simulink model "sm_wheel_loader_vehicle"  (R2025a)
settings: Solver=ode23t  StartTime=0.0  StopTime=70  RelTol=1e-3  AbsTol=1e-3  EnableMultiTasking=on
PostLoadFcn:
  | sm_wheel_loader_config_impl(bdroot,'Bucket')
StartFcn:
  | tic
StopFcn:
  | Elapsed_Sim_Time = toc;
  | disp(['Elapsed Sim Time = ' num2str(Elapsed_Sim_Time)]);
undefined symbols (not defined in the file or in its folder): Ideal, X, Y, Z
libraries: fl_lib x6, nesl_utility x5, sm_lib x4, sm_wheel_loader_lib x2, wheel_loader_contact_lib x2
Description:
  | Wheel Loader Chassis, Drivetrain, and Linkage
  | Copyright 2023-2025 The MathWorks, Inc.
settings Model: Creator=smiller  LastModifiedBy=smiller
settings SolverCC: AutoScaleAbsTol=off  AlgebraicLoopSolver=TrustRegion  MaxZcPerStep=1.0
settings DataIOCC: MaxDataPoints=10000  ReturnWorkspaceOutputs=off  SignalLoggingName=logsout_sm_wheel_loader_vehicle
settings OptimizationCC: ReuseModelBlockBuffer=off  LifeSpan=inf
settings DebuggingCC: UnconnectedInputMsg=warning  UnconnectedOutputMsg=warning  UnconnectedLineMsg=warning  AllowSymbolicDim=off  SubsystemReferenceDiagnosticForUnitTest=warning  SFUnexpectedBacktrackingDiag=warning  SFNoUnconditionalDefaultTransitionDiag=warning  SFExecutionAtInitializationDiag=none  ArithmeticOperatorsInVariantConditions=warning
settings ModelReferenceCC: EnableRefExpFcnMdlSchedulingChecks=on
settings SFSimCC: SimUseLocalCustomCode=off  CustomCodeUndefinedFunction=UseInterfaceOnly
settings RTWCC: RTWUseLocalCustomCode=off  GPUComputeCapability=3.5  DLArmComputeVersion=19.05
settings CodeAppCC: StateflowObjectComments=on
settings GRTTargetCC: TargetLangStandard=C89/C90 (ANSI)
settings ConfigComp: CovMetricSettings=dw  CovSaveCumulativeToWorkspaceVar=on  CovSaveSingleToWorkspaceVar=on  CovExternalEMLEnable=off  CovSFcnEnable=off
settings SimscapeCC: SimscapeLogType=all  SimscapeLogSimulationStatistics=on  SimscapeLogName=simlog_sm_wheel_loader_vehicle  SimscapeLogLimitData=off  SimscapeLogDataHistory=10000.0
settings DiagnosticsConfigSet: SimMechanicsUnconnectedFramePorts=none  SimMechanicsConflictingReferenceFrames=none
settings ExplorerConfigSet: InternalSimMechanicsExplorerSettings="<ExplorerConfiguration><canonicalview>default</canonicalview><AnimationSetting><BasePlaybackSpeed>1.0</BasePlaybackSpeed><PlaybackSpeedFactor>4.0</PlaybackSpeedFactor></AnimationSetting><TilePanel><TileInfo><Tiles Columns=\"2\" Count=\"3\" Rows=\"2\"><Column Weight=\"0.5\"/><Column Weight=\"0.5\"/><Row Weight=\"0.5\"/><Row Weight=\"0.5\"/><Tile Height=\"2\" Width=\"1\" X=\"0\" Y=\"0\"/><Tile Height=\"1\" Width=\"1\" X=\"1\" Y=\"0\"/><Tile Height=\"1\" Width=\"1\" X=\"1\" Y=\"1\"/></Tiles></TileInfo><SceneInfo><SceneViewer><BGColor><R>1</R><G>1</G><B>1</B></BGColor><Camera><DoPerspective>off</DoPerspective><Position><X>-0.569412591350047403</X><Y>-3.41040347859815096</Y><Z>11.8871003431686244</Z></Position><Center><X>-0.569412591350047403</X><Y>-3.41040347859815096</Y><Z>1.14793638608369264</Z></Center><Up><X>0</X><Y>1</Y><Z>-0</Z></Up><ViewLimDist>1</ViewLimDist><YLim>8.07680835846142919</YLim><XLim>8.82649459838867223</XLim></Camera></SceneViewer><SceneViewer><BGColor><R>1</R><G>1</G><B>1</B></BGColor><Camera><DoPerspective>on</DoPerspective><Position><X>1.34928960365821002e-16</X><Y>1.6204999999999985</Y><Z>1.58342999999999989</Z></Position><Center><X>8.83082669489443361e-17</X><Y>0.620499999999998497</Y><Z>1.58343000000000012</Z></Center><Up><X>0</X><Y>0</Y><Z>1</Z></Up><ViewLimDist>1</ViewLimDist><YLim>0.466307658154998583</YLim><XLim>1.0355017035185734</XLim></Camera></SceneViewer><SceneViewer><BGColor><R>1</R><G>1</G><B>1</B></BGColor><Camera><DoPerspective>on</DoPerspective><Position><X>-4.09999999999999964</X><Y>-0.0795000000000013474</Y><Z>1.08343000000000012</Z></Position><Center><X>-3.09999999999999964</X><Y>-0.079500000000001389</Y><Z>1.08343000000000012</Z></Center><Up><X>0</X><Y>0</Y><Z>1</Z></Up><ViewLimDist>1</ViewLimDist><YLim>0.466307658154998583</YLim><XLim>1.0355017035185734</XLim></Camera></SceneViewer></SceneInfo></TilePanel><MechEditorPanel><Cameras><Camera><Id>Camera2</Id><Value><Name>Track_FrameR_DiffR_toR</Name><NativeCamera><PositionTrackingFeature>Wheel_Loader.Vehicle.Frame_Rear.Camera_Frames.Reference_Camera_DiffR_toR.R</PositionTrackingFeature><CenterTrackingFeature>Wheel_Loader.Vehicle.Frame_Rear.Camera_Frames.Reference_Camera_DiffR_toR.R</CenterTrackingFeature><UpVectorTrackingFeature>Wheel_Loader.Vehicle.Frame_Rear.Camera_Frames.Reference_Camera_DiffR_toR.R</UpVectorTrackingFeature><CenterTrackingOrigin>off</CenterTrackingOrigin><CenterTrackingDirection>-Y</CenterTrackingDirection><UpVectorTrackingDirection>+Z</UpVectorTrackingDirection></NativeCamera></Value></Camera><Camera><Id>Camera3</Id><Value><Name>Track_FrameR_FinalDriveRR</Name><NativeCamera><PositionTrackingFeature>Wheel_Loader.Vehicle.Frame_Rear.Camera_Frames.Reference_Camera_FinalDriveRR.R</PositionTrackingFeature><CenterTrackingFeature>Wheel_Loader.Vehicle.Frame_Rear.Camera_Frames.Reference_Camera_FinalDriveRR.R</CenterTrackingFeature><UpVectorTrackingFeature>Wheel_Loader.Vehicle.Frame_Rear.Camera_Frames.Reference_Camera_FinalDriveRR.R</UpVectorTrackingFeature><CenterTrackingOrigin>off</CenterTrackingOrigin><CenterTrackingDirection>-X</CenterTrackingDirection><UpVectorTrackingDirection>+Z</UpVectorTrackingDirection></NativeCamera></Value></Camera><Camera><Id>Camera4</Id><Value><Name>Track_FrameR_Right</Name><NativeCamera><PositionTrackingFeature>Wheel_Loader.Vehicle.Frame_Rear.Camera_Frames.Reference_Camera_Right.R</PositionTrackingFeature><CenterTrackingFeature>Wheel_Loader.Vehicle.Frame_Rear.Camera_Frames.Reference_Camera_Right.R</CenterTrackingFeature><UpVectorTrackingFeature>Wheel_Loader.World_Frame.W</UpVectorTrackingFeature><CenterTrackingOrigin>off</CenterTrackingOrigin><CenterTrackingDirection>-X</CenterTrackingDirection><UpVectorTrackingDirection>+Z</UpVectorTrackingDirection></NativeCamera></Value></Camera><Camera><Id>Camera5</Id><Value><Name>Track_FrameR_Cab</Name><NativeCamera><PositionTrackingFeature>Wheel_Loader.Vehicle.Frame_Rear.Camera_Frames.Reference_Camera_Cab.R</PositionTrackingFeature><CenterTrackingFeature>Wheel_Loader.Vehicle.Frame_Rear.Camera_Frames.Reference_Camera_Cab.R</CenterTrackingFeature><UpVectorTrackingFeature>Wheel_Loader.World_Frame.W</UpVectorTrackingFeature><CenterTrackingOrigin>off</CenterTrackingOrigin><CenterTrackingDirection>+Y</CenterTrackingDirection><UpVectorTrackingDirection>+Z</UpVectorTrackingDirection></NativeCamera></Value></Camera><Camera><Id>Camera6</Id><Value><Name>Track_FrameR_RR</Name><NativeCamera><PositionTrackingFeature>Wheel_Loader.Vehicle.Frame_Rear.Camera_Frames.Reference_Camera_RR.R</PositionTrackingFeature><CenterTrackingFeature>Wheel_Loader.Vehicle.Frame_Rear.Camera_Frames.Reference_Camera_RR.R</CenterTrackingFeature><UpVectorTrackingFeature>Wheel_Loader.World_Frame.W</UpVectorTrackingFeature><CenterTrackingOrigin>off</CenterTrackingOrigin><CenterTrackingDirection>+X</CenterTrackingDirection><UpVectorTrackingDirection>+Z</UpVectorTrackingDirection></NativeCamera></Value></Camera><Camera><Id>Camera7</Id><Value><Name>Track_FrameR_Rear</Name><NativeCamera><PositionTrackingFeature>Wheel_Loader.Vehicle.Frame_Rear.Camera_Frames.Reference_Camera_Rear.R</PositionTrackingFeature><CenterTrackingFeature>Wheel_Loader.Vehicle.Frame_Rear.Camera_Frames.Reference_Camera_Rear.R</CenterTrackingFeature><UpVectorTrackingFeature>Wheel_Loader.World_Frame.W</UpVectorTrackingFeature><CenterTrackingOrigin>off</CenterTrackingOrigin><CenterTrackingDirection>+Y</CenterTrackingDirection><UpVectorTrackingDirection>+Z</UpVectorTrackingDirection></NativeCamera></Value></Camera><Camera><Id>Camera8</Id><Value><Name>Track_FrameF_RR</Name><NativeCamera><PositionTrackingFeature>Wheel_Loader.Vehicle.Frame_Front.Camera_Frames.Reference_Camera_RR.R</PositionTrackingFeature><CenterTrackingFeature>Wheel_Loader.Vehicle.Frame_Front.Camera_Frames.Reference_Camera_RR.R</CenterTrackingFeature><UpVectorTrackingFeature>Wheel_Loader.Vehicle.Frame_Front.Camera_Frames.Reference_Camera_RR.R</UpVectorTrackingFeature><CenterTrackingOrigin>off</CenterTrackingOrigin><CenterTrackingDirection>+X</CenterTrackingDirection><UpVectorTrackingDirection>+Z</UpVectorTrackingDirection></NativeCamera></Value></Camera><Camera><Id>Camera9</Id><Value><Name>Track_FrameF_ImplRR</Name><NativeCamera><PositionTrackingFeature>Wheel_Loader.Vehicle.Frame_Front.Camera_Frames.Reference_Camera_ImplRR.R</PositionTrackingFeature><CenterTrackingFeature>Wheel_Loader.Vehicle.Frame_Front.Camera_Frames.Reference_Camera_ImplRR.R</CenterTrackingFeature><UpVectorTrackingFeature>Wheel_Loader.Vehicle.Frame_Front.Camera_Frames.Reference_Camera_ImplRR.R</UpVectorTrackingFeature><CenterTrackingOrigin>off</CenterTrackingOrigin><CenterTrackingDirection>+X</CenterTrackingDirection><UpVectorTrackingDirection>+Z</UpVectorTrackingDirection></NativeCamera></Value></Camera><Camera><Id>Camera10</Id><Value><Name>Track_FrameF_Roof</Name><NativeCamera><PositionTrackingFeature>Wheel_Loader.Vehicle.Frame_Front.Camera_Frames.Reference_Camera_Roof.R</PositionTrackingFeature><CenterTrackingFeature>Wheel_Loader.Vehicle.Frame_Front.Camera_Frames.Reference_Camera_Roof.R</CenterTrackingFeature><UpVectorTrackingFeature>Wheel_Loader.Vehicle.Frame_Front.Camera_Frames.Reference_Camera_Roof.R</UpVectorTrackingFeature><CenterTrackingOrigin>off</CenterTrackingOrigin><CenterTrackingDirection>+Y</CenterTrackingDirection><UpVectorTrackingDirection>+Z</UpVectorTrackingDirection></NativeCamera></Value></Camera><Camera><Id>Camera11</Id><Value><Name>Track_FrameR_Driveline_RR</Name><NativeCamera><PositionTrackingFeature>Wheel_Loader.Vehicle.Frame_Rear.Camera_Frames.Reference_Camera_Driveline_RR.R</PositionTrackingFeature><CenterTrackingFeature>Wheel_Loader.Vehicle.Frame_Rear.Camera_Frames.Reference_Camera_Driveline_RR.R</CenterTrackingFeature><UpVectorTrackingFeature>Wheel_Loader.Vehicle.Frame_Rear.Camera_Frames.Reference_Camera_Driveline_RR.R</UpVectorTrackingFeature><CenterTrackingOrigin>off</CenterTrackingOrigin><CenterTrackingDirection>+Y</CenterTrackingDirection><UpVectorTrackingDirection>+Z</UpVectorTrackingDirection></NativeCamera></Value></Camera><Camera><Id>Camera12</Id><Value><Name>Track_FrameR_Driveline_Top</Name><NativeCamera><PositionTrackingFeature>Wheel_Loader.Vehicle.Frame_Rear.Camera_Frames.Reference_Camera_Driveline_Top.R</PositionTrackingFeature><CenterTrackingFeature>Wheel_Loader.Vehicle.Frame_Rear.Camera_Frames.Reference_Camera_Driveline_Top.R</CenterTrackingFeature><UpVectorTrackingFeature>Wheel_Loader.Vehicle.Frame_Rear.Camera_Frames.Reference_Camera_Driveline_Top.R</UpVectorTrackingFeature><CenterTrackingOrigin>off</CenterTrackingOrigin><CenterTrackingDirection>-Z</CenterTrackingDirection><UpVectorTrackingDirection>-X</UpVectorTrackingDirection></NativeCamera></Value></Camera><Camera><Id>Camera13</Id><Value><Name>Track_FrameR_Driveline_Top_FixO</Name><NativeCamera><PositionTrackingFeature>Wheel_Loader.Vehicle.Frame_Rear.Camera_Frames.Reference_Camera_Driveline_Top.R</PositionTrackingFeature><CenterTrackingFeature>Wheel_Loader.Vehicle.Frame_Rear.Camera_Frames.Reference_Camera_Driveline_Top.R</CenterTrackingFeature><UpVectorTrackingFeature>Wheel_Loader.World_Frame.W</UpVectorTrackingFeature><CenterTrackingOrigin>off</CenterTrackingOrigin><CenterTrackingDirection>-Z</CenterTrackingDirection><UpVectorTrackingDirection>+X</UpVectorTrackingDirection></NativeCamera></Value></Camera><Camera><Id>Camera14</Id><Value><Name>Track_FrameR_DiffR_toF</Name><NativeCamera><PositionTrackingFeature>Wheel_Loader.Vehicle.Frame_Rear.Camera_Frames.Reference_Camera_DiffR_toF.R</PositionTrackingFeature><CenterTrackingFeature>Wheel_Loader.Vehicle.Frame_Rear.Camera_Frames.Reference_Camera_DiffR_toF.R</CenterTrackingFeature><UpVectorTrackingFeature>Wheel_Loader.Vehicle.Frame_Rear.Camera_Frames.Reference_Camera_DiffR_toF.R</UpVectorTrackingFeature><CenterTrackingOrigin>off</CenterTrackingOrigin><CenterTrackingDirection>-Y</CenterTrackingDirection><UpVectorTrackingDirection>+Z</UpVectorTrackingDirection></NativeCamera></Value></Camera><Camera><Id>Camera15</Id><Value><Name>Track_FrameR_Driveline_Top_Low</Name><NativeCamera><PositionTrackingFeature>Wheel_Loader.Vehicle.Frame_Rear.Camera_Frames.Reference_Camera_Driveline_TopLow.R</PositionTrackingFeature><CenterTrackingFeature>Wheel_Loader.Vehicle.Frame_Rear.Camera_Frames.Reference_Camera_Driveline_TopLow.R</CenterTrackingFeature><UpVectorTrackingFeature>Wheel_Loader.Vehicle.Frame_Rear.Camera_Frames.Reference_Camera_Driveline_TopLow.R</UpVectorTrackingFeature><CenterTrackingOrigin>off</CenterTrackingOrigin><CenterTrackingDirection>-Z</CenterTrackingDirection><UpVectorTrackingDirection>-X</UpVectorTrackingDirection></NativeCamera></Value></Camera><Camera><Id>Camera16</Id><Value><Name>Track_FrameF_LinkageR</Name><NativeCamera><PositionTrackingFeature>Wheel_Loader.Vehicle.Frame_Front.Camera_Frames.Transform_Camera_LinkageR.F</PositionTrackingFeature><CenterTrackingFeature>Wheel_Loader.Vehicle.Frame_Front.Camera_Frames.Transform_Camera_LinkageR.F</CenterTrackingFeature><UpVectorTrackingFeature>Wheel_Loader.Vehicle.Frame_Front.Camera_Frames.Transform_Camera_LinkageR.F</UpVectorTrackingFeature><CenterTrackingOrigin>off</CenterTrackingOrigin><CenterTrackingDirection>-X</CenterTrackingDirection><UpVectorTrackingDirection>+Z</UpVectorTrackingDirection></NativeCamera></Value></Camera><Camera><Id>Camera17</Id><Value><Name>TrackF_WheelFR</Name><NativeCamera><PositionTrackingFeature>Wheel_Loader.Vehicle.Frame_Front.Camera_Frames.Reference_Camera_WhlFR.R</PositionTrackingFeature><CenterTrackingFeature>Wheel_Loader.Vehicle.Frame_Front.Camera_Frames.Reference_Camera_WhlFR.R</CenterTrackingFeature><UpVectorTrackingFeature>Wheel_Loader.World_Frame.W</UpVectorTrackingFeature><CenterTrackingOrigin>off</CenterTrackingOrigin><CenterTrackingDirection>-X</CenterTrackingDirection><UpVectorTrackingDirection>+Z</UpVectorTrackingDirection></NativeCamera></Value></Camera><Camera><Id>Camera18</Id><Value><Name>TrackF_IsoFR</Name><NativeCamera><PositionTrackingFeature>Wheel_Loader.Vehicle.Frame_Front.Camera_Frames.Reference_Camera_IsoFR.R</PositionTrackingFeature><CenterTrackingFeature>Wheel_Loader.Vehicle.Frame_Front.Camera_Frames.Reference_Camera_IsoFR.R</CenterTrackingFeature><UpVectorTrackingFeature>Wheel_Loader.World_Frame.W</UpVectorTrackingFeature><CenterTrackingOrigin>off</CenterTrackingOrigin><CenterTrackingDirection>-X</CenterTrackingDirection><UpVectorTrackingDirection>+Z</UpVectorTrackingDirection></NativeCamera></Value></Camera></Cameras><GfxPanelCameraMap><MapElement CameraMLId=\"Camera5\" GfxPanelIndex=\"1\"/><MapElement CameraMLId=\"Camera4\" GfxPanelIndex=\"2\"/></GfxPanelCameraMap><VideoCreator><PlaybackSpeedRatio>1</PlaybackSpeedRatio><FrameRate>30</FrameRate><VideoFormat>MPEG-4</VideoFormat><FrameSize>auto</FrameSize></VideoCreator></MechEditorPanel></ExplorerConfiguration>"

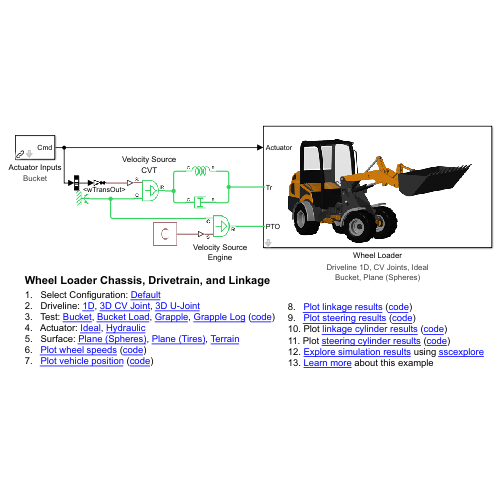
[thumbnail: Simulink's stored preview of the top-level diagram]
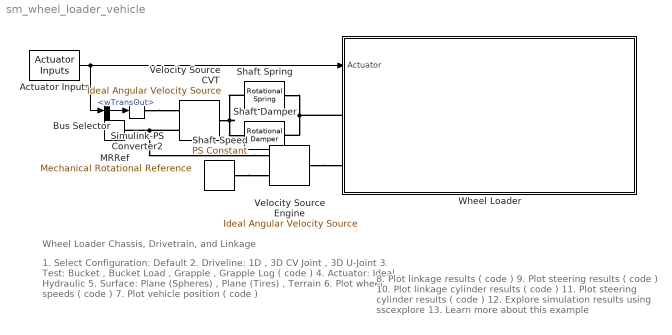
== system sm_wheel_loader_vehicle ==
  note: Wheel Loader Chassis, Drivetrain, and Linkage
  note: 1. Select Configuration: Default
      | 2. Driveline: 1D , 3D CV Joint , 3D U-Joint
      | 3. Test: Bucket , Bucket Load , Grapple , Grapple Log ( code )
      | 4. Actuator: Ideal , Hydraulic
      | 5. Surface: Plane (Spheres) , Plane (Tires) , Terrain
      | 6. Plot wheel speeds ( code )
      | 7. Plot vehicle position ( code )
  note: 8. Plot linkage results ( code )
      | 9. Plot steering results ( code )
      | 10. Plot linkage cylinder results ( code )
      | 11. Plot steering cylinder results ( code )
      | 12. Explore simulation results using sscexplore
      | 13. Learn more about this example
  Actuator Inputs : sm_wheel_loader_lib/Actuator Inputs  popup_steering=on  popup_linkage=on  popup_impl=Bucket
      settings: AttributesFormatString=%<popup_impl>
  Bus Selector : BusSelector  OutputSignals=Operator.wTransOut
  MRRef : fl_lib/Mechanical/Rotational Elements/Mechanical Rotational Reference
  Shaft Damper : fl_lib/Mechanical/Rotational Elements/Rotational Damper  D=5 N*m*s/rad  w_specify=off  w_priority=None  w=0 rad/s  w_nominal_specify=off  w_nominal_value=1  w_nominal_unit=rad/s  t_specify=off  t_priority=None  t=0 N*m  t_nominal_specify=off  t_nominal_value=1  t_nominal_unit=N*m
  Shaft Speed : fl_lib/Physical Signals/Sources/PS Constant  constant=HMPST.Eng.wTarget rpm
  Shaft Spring : fl_lib/Mechanical/Rotational Elements/Rotational Spring  spr_rate=1000 N*m/rad  w_specify=off  w_priority=None  w=0 rad/s  w_nominal_specify=off  w_nominal_value=1  w_nominal_unit=rad/s  t_specify=off  t_priority=None  t=0 N*m  t_nominal_specify=off  t_nominal_value=1  t_nominal_unit=N*m  phi_specify=off  phi_priority=High  phi=0 rad  phi_nominal_specify=off  phi_nominal_value=1  phi_nominal_unit=rad
  Simulink-PS Converter2 : nesl_utility/Simulink-PS Converter  PhysicalDomain=network_engine_domain  SubClassName=ps_input  LeftPortType=input  RightPortType=output  PseudoPeriodic=off  Frequencies=[]  NoiseDistribution=none  NoiseParameters=[]  Unit=rpm  AffineConversion=off  FilteringAndDerivatives=filter  SimscapeFilterOrder=2  InputFilterTimeConstant=0.1  UdotUserProvided=0
  Velocity Source CVT : fl_lib/Mechanical/Mechanical Sources/Ideal Angular Velocity Source
  Velocity Source Engine : fl_lib/Mechanical/Mechanical Sources/Ideal Angular Velocity Source
  Wheel Loader : Subsystem  mask(Wheel Loader Vehicle and Load){popup_surface=Plane (Spheres), popup_impl=Bucket, popup_actuator_model=Ideal, popup_driveline=1D, CV Joints}
      mask prompts: popup_surface "Surface"; popup_impl "Implement"; popup_actuator_model "Actuator Model"; popup_driveline "Driveline"
      mask help: Models chassis, driveline, and linkage for a wheel loader. Includes configurable model of load. Use drop down menus to configure system options.
      mask init:
      | if(popup_surface==1)
      |     set_param([gcb '/Surface'],'LabelModeActiveChoice','Plane')
      |     set_param([gcb '/Vehicle'],'popup_contact','Sphere')
      | elseif(popup_surface==2)
      |     set_param([gcb '/Surface'],'LabelModeActiveChoice','Plane')
      |     set_param([gcb '/Vehicle'],'popup_contact','Tire')
      | elseif(popup_surface==3)
      |     set_param([gcb '/Surface'],'LabelModeActiveChoice','Terrain')
      |     set_param([gcb '/Vehicle'],'popup_contact','Points')
      | end
      | if(popup_impl==1)
      |     set_param([gcb '/Vehicle'],'popup_impl','Bucket')
      |     set_param([gcb '/Vehicle'],'popup_load','None')
      | elseif(popup_impl==2)
      |     set_param([gcb '/Vehicle'],'popup_impl','Bucket')
      |     set_param([gcb '/Vehicle'],'popup_load','Inertia')
      | elseif(popup_impl==3)
      |     set_param([gcb '/Vehicle'],'popup_impl','Grapple')
      |     set_param([gcb '/Vehicle'],'popup_load','None')
      | elseif(popup_impl==4)
      |     set_param([gcb '/Vehicle'],'popup_impl','Grapple')
      |     set_param([gcb '/Vehicle'],'popup_load','Log')
      | end
      | if(popup_driveline==1)
      |     set_param([gcb '/Vehicle'],'popup_driveline_model','Driveline 1D')
      |     set_param([gcb '/Vehicle'],'popup_driveJointF','CV Joint')
      |     set_param([gcb '/Vehicle'],'popup_driveJointR','CV Joint')
      | elseif(popup_driveline==2)
      |     set_param([gcb '/Vehicle'],'popup_driveline_model','Driveline 3D')
      |     set_param([gcb '/Vehicle'],'popup_driveJointF','CV Joint')
      |     set_param([gcb '/Vehicle'],'popup_driveJointR','CV Joint')
      | elseif(popup_driveline==3)
      |     set_param([gcb '/Vehicle'],'popup_driveline_model','Driveline 3D')
      |     set_param([gcb '/Vehicle'],'popup_driveJointF','U Joint')
      |     set_param([gcb '/Vehicle'],'popup_driveJointR','U Joint')
      | end
      settings: AttributesFormatString=|
      | Driveline %<popup_driveline>, %<popup_actuator_model>
      | %<popup_impl>, %<popup_surface>
      mask TypeOptions popup_surface: Plane (Spheres) | Plane (Tires) | Terrain
      mask TypeOptions popup_impl: Bucket | Bucket Load | Grapple | Grapple Log
      mask TypeOptions popup_actuator_model: Vehicle/popup_actuator_model
      mask TypeOptions popup_driveline: 1D, CV Joints | 3D, CV Joints | 3D, U Joints
      mask Display: image('sm_wheel_loader_vehicle_IMAGE.png');
  wires:
  Bus Selector/1 -> Simulink-PS Converter2/1  "<wTransOut>"
  Actuator Inputs/1 -> Bus Selector/1, Wheel Loader/1(Actuator)
  connections:
  Shaft Spring/RConn1 -- Shaft Damper/RConn1 -- Velocity Source CVT/LConn1
  Velocity Source Engine/RConn2 -- MRRef/LConn1 -- Velocity Source CVT/RConn2
  Simulink-PS Converter2/RConn1 -- Velocity Source CVT/RConn1
  Shaft Spring/LConn1 -- Wheel Loader/LConn1 -- Shaft Damper/LConn1
  Shaft Speed/RConn1 -- Velocity Source Engine/RConn1
  Velocity Source Engine/LConn1 -- Wheel Loader/LConn2

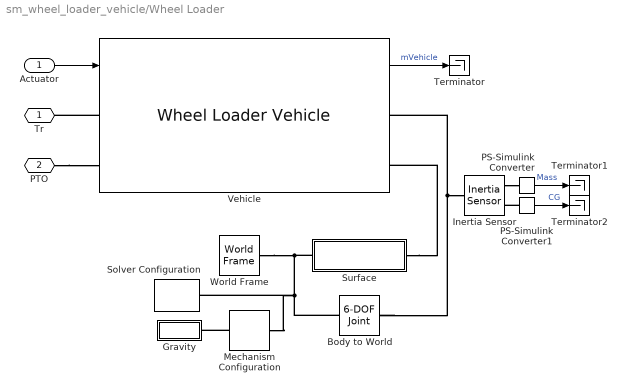
== system sm_wheel_loader_vehicle/Wheel Loader ==
  Actuator : Inport
  Body to World : sm_lib/Joints/6-DOF Joint  JointMode=Normal  CompositeWrenchDir=FollowerOnBase  CompositeWrenchFrame=BaseFrame  SenseConstraintForce=off  SenseConstraintTorque=off  SenseTotalForce=off  SenseTotalTorque=off  PxPositionTargetSpecify=off  PxPositionTargetPriority=High  PxPositionTargetValue=0  PxPositionTargetValueUnits=m  PxVelocityTargetSpecify=off  PxVelocityTargetPriority=High  PxVelocityTargetValue=0  PxVelocityTargetValueUnits=m/s  PxEquilibriumPosition=0  PxEquilibriumPositionUnits=m  PxSpringStiffness=0  PxSpringStiffnessUnits=N/m  PxDampingCoefficient=0  PxDampingCoefficientUnits=N/(m/s)  PxLowerLimitSpecify=off  PxLowerLimitBound=-1  PxLowerLimitBoundUnits=m  PxLowerLimitStiffness=1e6  PxLowerLimitStiffnessUnits=N/m  PxLowerLimitDamping=1e3  PxLowerLimitDampingUnits=N/(m/s)  PxLowerLimitTransitionRegionWidth=1e-4  PxLowerLimitTransitionRegionWidthUnits=m  PxUpperLimitSpecify=off  PxUpperLimitBound=1  PxUpperLimitBoundUnits=m  PxUpperLimitStiffness=1e6  PxUpperLimitStiffnessUnits=N/m  PxUpperLimitDamping=1e3  PxUpperLimitDampingUnits=N/(m/s)  PxUpperLimitTransitionRegionWidth=1e-4  PxUpperLimitTransitionRegionWidthUnits=m  PxTorqueActuationMode=NoTorque  PxMotionActuationMode=ComputedMotion  PxSensePosition=off  PxSenseVelocity=off  PxSenseAcceleration=off  PxSenseTorqueForce=off  PxSenseLowerLimitTorqueForce=off  PxSenseUpperLimitTorqueForce=off  PyPositionTargetSpecify=off  PyPositionTargetPriority=High  PyPositionTargetValue=0  PyPositionTargetValueUnits=m  PyVelocityTargetSpecify=off  PyVelocityTargetPriority=High  PyVelocityTargetValue=0  PyVelocityTargetValueUnits=m/s  PyEquilibriumPosition=0  PyEquilibriumPositionUnits=m  PySpringStiffness=0  PySpringStiffnessUnits=N/m  PyDampingCoefficient=0  PyDampingCoefficientUnits=N/(m/s)  PyLowerLimitSpecify=off  PyLowerLimitBound=-1  PyLowerLimitBoundUnits=m  PyLowerLimitStiffness=1e6  PyLowerLimitStiffnessUnits=N/m  PyLowerLimitDamping=1e3  PyLowerLimitDampingUnits=N/(m/s)  PyLowerLimitTransitionRegionWidth=1e-4  PyLowerLimitTransitionRegionWidthUnits=m  PyUpperLimitSpecify=off  PyUpperLimitBound=1  PyUpperLimitBoundUnits=m  PyUpperLimitStiffness=1e6  PyUpperLimitStiffnessUnits=N/m  PyUpperLimitDamping=1e3  PyUpperLimitDampingUnits=N/(m/s)  PyUpperLimitTransitionRegionWidth=1e-4  PyUpperLimitTransitionRegionWidthUnits=m  PyTorqueActuationMode=NoTorque  PyMotionActuationMode=ComputedMotion  PySensePosition=off  PySenseVelocity=off  PySenseAcceleration=off  PySenseTorqueForce=off  PySenseLowerLimitTorqueForce=off  PySenseUpperLimitTorqueForce=off  PzPositionTargetSpecify=on  PzPositionTargetPriority=High  PzPositionTargetValue=0  PzPositionTargetValueUnits=m  PzVelocityTargetSpecify=off  PzVelocityTargetPriority=High  PzVelocityTargetValue=0  PzVelocityTargetValueUnits=m/s  PzEquilibriumPosition=0  PzEquilibriumPositionUnits=m  PzSpringStiffness=0  PzSpringStiffnessUnits=N/m  PzDampingCoefficient=0  PzDampingCoefficientUnits=N/(m/s)  PzLowerLimitSpecify=off  PzLowerLimitBound=-1  PzLowerLimitBoundUnits=m  PzLowerLimitStiffness=1e6  PzLowerLimitStiffnessUnits=N/m  PzLowerLimitDamping=1e3  PzLowerLimitDampingUnits=N/(m/s)  PzLowerLimitTransitionRegionWidth=1e-4  PzLowerLimitTransitionRegionWidthUnits=m  PzUpperLimitSpecify=off  PzUpperLimitBound=1  PzUpperLimitBoundUnits=m  PzUpperLimitStiffness=1e6  PzUpperLimitStiffnessUnits=N/m  PzUpperLimitDamping=1e3  PzUpperLimitDampingUnits=N/(m/s)  PzUpperLimitTransitionRegionWidth=1e-4  PzUpperLimitTransitionRegionWidthUnits=m  PzTorqueActuationMode=NoTorque  PzMotionActuationMode=ComputedMotion  PzSensePosition=off  PzSenseVelocity=off  PzSenseAcceleration=off  PzSenseTorqueForce=off  PzSenseLowerLimitTorqueForce=off  PzSenseUpperLimitTorqueForce=off  SphPositionTargetSpecify=on  SphPositionTargetPriority=High  SphPositionTargetRotationMethod=StandardAxis  SphPositionTargetFollAlignAxisA=+X  SphPositionTargetBaseAlignAxisA=+Y  SphPositionTargetFollAlignAxisB=+Y  SphPositionTargetBaseAlignAxisB=+Z  SphPositionTargetRotationStandardAxis=+Z  SphPositionTargetRotationAngle=-90  SphPositionTargetRotationAngleUnits=deg  SphPositionTargetRotationArbitraryAxis=[0 0 1]  SphPositionTargetRotationSequenceAxes=FollowerAxes  SphPositionTargetRotationSequence=XYX  SphPositionTargetRotationSequenceAngles=[0 0 0]  SphPositionTargetRotationSequenceAnglesUnits=deg  SphPositionTargetRotationMatrix=[1 0 0; 0 1 0; 0 0 1]  SphPositionTargetQuaternion=[1 0 0 0]  SphVelocityTargetSpecify=off  SphVelocityTargetPriority=High  SphVelocityTargetValue=[0 0 0]  SphVelocityTargetValueUnits=deg/s  SphVelocityTargetInFollowerFrame=on  SphEqPosRotationMethod=None  SphEqPosFollAlignAxisA=+X  SphEqPosBaseAlignAxisA=+Y  SphEqPosFollAlignAxisB=+Y  SphEqPosBaseAlignAxisB=+Z  SphEqPosRotationStandardAxis=+Z  SphEqPosRotationAngle=0.0  SphEqPosRotationAngleUnits=deg  SphEqPosRotationArbitraryAxis=[0 0 1]  SphEqPosRotationSequenceAxes=FollowerAxes  SphEqPosRotationSequence=XYX  SphEqPosRotationSequenceAngles=[0 0 0]  SphEqPosRotationSequenceAnglesUnits=deg  SphEqPosRotationMatrix=[1 0 0; 0 1 0; 0 0 1]  SphEqPosQuaternion=[1 0 0 0]  SphSpringStiffness=0  SphSpringStiffnessUnits=N*m/deg  SphDampingCoefficient=0  SphDampingCoefficientUnits=N*m/(deg/s)  SphLowerLimitSpecify=off  SphLowerLimitBound=15  SphLowerLimitBoundUnits=deg  SphLowerLimitStiffness=1e4  SphLowerLimitStiffnessUnits=N*m/deg  SphLowerLimitDamping=10  SphLowerLimitDampingUnits=N*m/(deg/s)  SphLowerLimitTransitionRegionWidth=0.1  SphLowerLimitTransitionRegionWidthUnits=deg  SphUpperLimitSpecify=off  SphUpperLimitBound=45  SphUpperLimitBoundUnits=deg  SphUpperLimitStiffness=1e4  SphUpperLimitStiffnessUnits=N*m/deg  SphUpperLimitDamping=10  SphUpperLimitDampingUnits=N*m/(deg/s)  SphUpperLimitTransitionRegionWidth=0.1  SphUpperLimitTransitionRegionWidthUnits=deg  SphTorqueActuationMode=NoTorque  SphActuateTorqueX=off  SphActuateTorqueY=off  SphActuateTorqueZ=off  SphActuateTorque=off  SphActuationFrame=BaseFrame  SphSensePosition=off  SphSenseVelocityX=off  SphSenseVelocityY=off  SphSenseVelocityZ=off  SphSenseVelocity=off  SphSenseAccelerationX=off  SphSenseAccelerationY=off  SphSenseAccelerationZ=off  SphSenseAcceleration=off  SphSenseLowerLimitTorqueMag=off  SphSenseUpperLimitTorqueMag=off  SphSensingFrame=BaseFrame
  Gravity : Subsystem
  Inertia Sensor : sm_lib/Body Elements/Inertia Sensor  SensorExtent=Mechanism  SpanWeldJoints=off  ExcludeGroundedBodies=on  MeasurementFrame=Attached  SenseMass=on  SenseCenterOfMass=on  SenseInertiaMatrix=off  SenseCenteredInertiaMatrix=off  SensePrincipalInertiaMatrix=off  SenseRotationMatrix=off  GraphicType=None  PrincipalInertiaFrameSize=20  GraphicVisPropType=SimpleVisualProperties  GraphicDiffuseColor=[0.5 0.5 0.5]  GraphicOpacity=1.0  GraphicSpecularColor=[0.5 0.5 0.5 1.0]  GraphicAmbientColor=[0.15 0.15 0.15 1.0]  GraphicEmissiveColor=[0.0 0.0 0.0 1.0]  GraphicShininess=75
  Mechanism Configuration : sm_lib/Utilities/Mechanism Configuration  UniformGravity=TimeVarying  GravityVector=[0 -9.80665 0]  GravityVectorUnits=m/s^2  LinearizationDelta=0.001  JointModeTransitionNonlinearIterations=2
  PS-Simulink Converter : nesl_utility/PS-Simulink Converter  PhysicalDomain=network_engine_domain  SubClassName=ps_output  LeftPortType=input  RightPortType=output  PseudoPeriodic=off  Frequencies=[]  VectorFormat=inherit  Unit=inherit  AffineConversion=off
  PS-Simulink Converter1 : nesl_utility/PS-Simulink Converter  PhysicalDomain=network_engine_domain  SubClassName=ps_output  LeftPortType=input  RightPortType=output  PseudoPeriodic=off  Frequencies=[]  VectorFormat=inherit  Unit=inherit  AffineConversion=off
  Solver Configuration : nesl_utility/Solver Configuration  PhysicalDomain=network_engine_domain  SubClassName=solver  LeftPortType=input  RightPortType=generic  Tones=[]  Harmonics=[]  SimulateNoise=off  Profile=off  UseLocalSampling=off  EnableSwitchedLinearOptims=on  FrequencyDomain=off  UseCCode=off  RelTol=0.001  AbsTol=0.001  MinStep=1e-09  ToWorkspace=off  RevertToSquareIcSolve=off  NumHomotopyIterations=100  PhasorMode=off  PhasorModeNumHarmonics=1  ConsistencySolver=NEWTON_XTOL_AFTER_FTOL  IndexReductionMethod=DerivativeReplacement  DoDC=off  ResidualTolerance=1e-09  ConsistencyTolSource=GLOBAL  ConsistencyAbsTol=0.001  ConsistencyRelTol=0.001  ConsistencyTolFactor=0.001  UseLocalSolver=off  LocalSolverChoice=NE_BACKWARD_EULER_ADVANCER  ResolveIndetEquations=on  FunctionEvalNumThread=1  LocalSolverSampleTime=0.001  DoFixedCost=off  MaxNonlinIter=3  MaxModeIter=2  ComputeImpulses=off  ImpulseIterations=2  LinearAlgebra=auto  LinearAlgebraNumThread=0  EquationFormulation=NE_TIME_EF  DelaysMemoryBudget=1024  AutomaticFiltering=on  FilteringTimeConstant=0.001  PartitionStorageMethod=AS_NEEDED  PartitionMemoryBudget=1024  PartitionMethod=ROBUST  MultibodyUseLocalSolver=off  MultibodyLocalSolverChoice=ODE1  MultibodyLocalSolverSampleTime=0.001
  Surface : Subsystem  Variant=on  VariantControlMode=label  VariantControl=Choice  LabelModeActiveChoice=Plane
  Terminator : Terminator
  Terminator1 : Terminator
  Terminator2 : Terminator
  Vehicle : sm_wheel_loader_lib/Wheel Loader Vehicle  VariantControl=simVariant == 1  popup_impl=Bucket  popup_actuator_model=Ideal  popup_load=None  popup_driveline_model=Driveline 1D  popup_driveJointF=CV Joint  popup_driveJointR=CV Joint  popup_contact=Sphere
      settings: AttributesFormatString=%<popup_driveline_model> (F: %<popup_driveJointF>, R: %<popup_driveJointR>), %<popup_impl> %<popup_load>, %<popup_contact>
  World Frame : sm_lib/Frames and Transforms/World Frame
  Tr : PMIOPort  Side=Left
  PTO : PMIOPort  Port=2  Side=Left
  wires:
  Vehicle/1 -> Terminator/1  "mVehicle"
  PS-Simulink Converter/1 -> Terminator1/1  "Mass"
  PS-Simulink Converter1/1 -> Terminator2/1  "CG"
  Actuator/1 -> Vehicle/1
  connections:
  Body to World/RConn1 -- Vehicle/RConn1 -- Inertia Sensor/LConn1
  Mechanism Configuration/RConn1 -- Solver Configuration/RConn1 -- World Frame/RConn1 -- Surface/LConn1 -- Body to World/LConn1
  Vehicle/LConn1 -- Tr/RConn1
  PTO/RConn1 -- Vehicle/LConn2
  Inertia Sensor/RConn1 -- PS-Simulink Converter/LConn1
  PS-Simulink Converter1/LConn1 -- Inertia Sensor/RConn2
  Surface/RConn1 -- Vehicle/RConn2
  Mechanism Configuration/LConn1 -- Gravity/RConn1

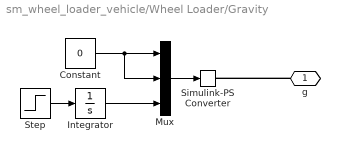
== system sm_wheel_loader_vehicle/Wheel Loader/Gravity ==
  Constant : Constant  Value=0
  Integrator : Integrator  LimitOutput=on  UpperSaturationLimit=0  LowerSaturationLimit=-9.81
  Mux : Mux  Inputs=3
  Simulink-PS Converter : nesl_utility/Simulink-PS Converter  PhysicalDomain=network_engine_domain  SubClassName=ps_input  LeftPortType=input  RightPortType=output  PseudoPeriodic=off  Frequencies=[]  NoiseDistribution=none  NoiseParameters=[]  Unit=1  AffineConversion=off  FilteringAndDerivatives=provide  SimscapeFilterOrder=1  InputFilterTimeConstant=0.001  UdotUserProvided=0
  Step : Step  Time=0.2  After=-9.81  SampleTime=0
  g : PMIOPort  Side=Right
  wires:
  Step/1 -> Integrator/1
  Constant/1 -> Mux/2, Mux/1
  Mux/1 -> Simulink-PS Converter/1
  Integrator/1 -> Mux/3
  connections:
  g/RConn1 -- Simulink-PS Converter/RConn1

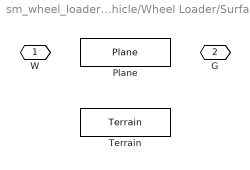
== system sm_wheel_loader_vehicle/Wheel Loader/Surface ==
  Plane : wheel_loader_contact_lib/Plane  VariantControl=Plane
  Terrain : wheel_loader_contact_lib/Terrain  VariantControl=Terrain
  W : PMIOPort  Side=Left
  G : PMIOPort  Port=2  Side=Right
